simulink model "something_even_dumber"  (R2026b)
settings: Solver=ode23t  StopTime=simulation.timeSim  MaxStep=1/(5*solarPlant.converterSwitchingFrequency)  AbsTol=1e-3
PreLoadFcn:
  | run('something_dumb.mlx');
values from neighbouring files (symbols this model uses):
  Csc = Csc_cell/Ns_sc*Np_sc    (= 200)    [LunarDAB_Params.m]
  eta_sc = 0.95    [LunarDAB_Params.m]
  fsw = 100e3    (= 100000)    [LunarDAB_Params.m]
  k_restore = 1    [LunarDAB_Params.m]
  kiCurrent = 2    [LunarDAB_Params.m]
  kiVoltage = 8    [LunarDAB_Params.m]
  kpCurrent = 0.005    [LunarDAB_Params.m]
  kpVoltage = 0.4    [LunarDAB_Params.m]
  lTotal = lSeries + Llk    [LunarDAB_Params.m]
  P170_Imp = im(ix)    [P170_PV_Initialize.m]
  P170_Vmp = vm(ix)    [P170_PV_Initialize.m]
  Rd_bat = dV_droop/Ibat_max    (= 0.232258064516)    [LunarDAB_Params.m]
  SC_enable = 1    [LunarDAB_Params.m]
  thetaMaxDab = pi/4    (= 0.785398163397)    [LunarDAB_Params.m]
  Tsw = 1/fsw    (= 1e-05)    [LunarDAB_Params.m]
  Vsc0 = sqrt((Vsc_max^2 + Vsc_min^2)/2)    [LunarDAB_Params.m]
  Vsc_max = 119    [LunarDAB_Params.m]
  Vsc_min = 66    [LunarDAB_Params.m]
undefined symbols (not defined in the file or in its folder): a_lpf_sys, battery, bms, connectedLoad, dcVoltage, eta_dab, Ibat_sign, lunarCase, maxSoC, maxVdc, minIrrad, minSoC, minVdc, Ndab, olTime, P170_T, sc, sensor, solarPlant
libraries: nesl_utility x13, fl_lib x12, simulink x7, slpidlib x2, batteryecm_lib x1, simulink_extras x1, ee_lib x1
settings Model: Creator=The MathWorks, Inc.  LastModifiedBy=aj26g
settings SolverCC: AutoScaleAbsTol=off
settings DataIOCC: DSMLogging=off  ReturnWorkspaceOutputs=off  SaveOutput=off  SaveTime=off  SignalLoggingName=SolarPVDCWithBattery_logDB
settings OptimizationCC: ReuseModelBlockBuffer=off
settings DebuggingCC: SymbolicDimsDataTypeCodeGenerationDiagnostic=none  UnderSpecifiedDimensionMsg=warning
settings SFSimCC: CustomCodeUndefinedFunction=UseInterfaceOnly
settings RTWCC: DLArmComputeVersion=19.05
settings SimscapeCC: SimscapeLogName=simlog_SolarPVDCWithBattery  SimscapeLogSimulationStatistics=on  SimscapeLogType=all  SimscapeUseEnergyAccounting=off

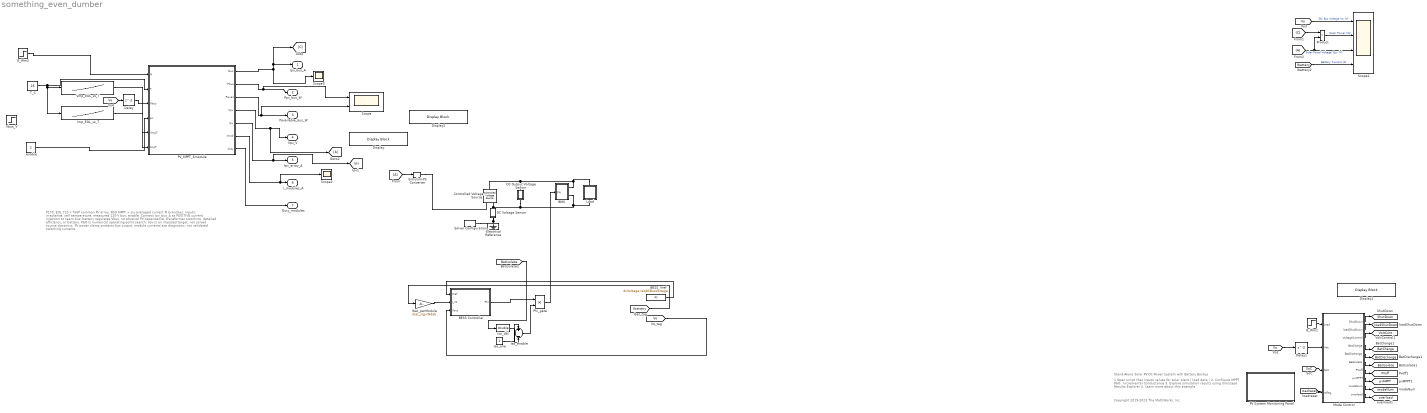
== system something_even_dumber ==
  note: 1 Open script that inputs values for solar plant ( load data )
      | 2. Configure MPPT P&O , Incremental Conductance
      | 3. Explore simulation results using Simscape Results Explorer
      | 4. Learn more about this example
  note: Stand-Alone Solar PV DC Power System with Battery Backup
  note: Copyright 2019-2023 The MathWorks, Inc.
  note: P170: EOL 72S x 756P common PV array. P&O MPPT + six averaged current PI branches.
      | Inputs: irradiance, cell temperature, measured 120-V bus, enable.
      | Connect Ipv_bus_A as POSITIVE current injection to team bus; battery regulates Vbus.
      |
      | no physical PV capacitance, transformer switching, detailed efficiency, or battery.
      | P&O is numerical operating-point search; Vpv is an imposed target, not solved source dynamics.
      | PV power clamp protects bus output; module currents are diagnostic, not validated switching currents.
  BESS Controller : Subsystem
  BESS_Vref : Constant  Value=dcVoltage.reqDCBusVoltage
  BMS : Subsystem
  Controlled Voltage Source : fl_lib/Electrical/Electrical Sources/Controlled Voltage Source
  DC Output Voltage Sensor : Subsystem
      mask Display: disp('v')
  DC Voltage Sensor : Subsystem
      mask Display: disp('v');
  Delay : Delay
  Delay1 : Delay
  Display : DisplayBlock  LabelPosition=Hide  Transparency=1  GridColor=[0.502, 0.502, 0.502]
  Display1 : DisplayBlock  LabelPosition=Hide  Transparency=1  GridColor=[0.502, 0.502, 0.502]
  Display2 : DisplayBlock  LabelPosition=Hide  Transparency=1  GridColor=[0.502, 0.502, 0.502]
  Electrical Reference : fl_lib/Electrical/Electrical Elements/Electrical Reference
  From : From
  From2 : From
  G_Wm1 : Step  Time=0.8  InitialValue=1367  FinalValue=700  SampleTime=0
  G_Wm2 : Step  Time=0.8  InitialValue=1367  FinalValue=700  SampleTime=0
  Goto2 : Goto
  Ibat_perModule : Gain  Gain=Ibat_sign/Ndab
  Imp_EOL_vs_T : Lookup_n-D  NumberOfTableDimensions=1  BreakpointsForDimension1=P170_T  Table=P170_Imp  InternalRulePriority=Speed  RndMeth=Simplest
  Iso_dbl : DataTypeConversion  OutDataTypeStr=double  SaturateOnIntegerOverflow=off  RndMeth=Floor
  Iso_enable : Sum  Inputs=+-
  Iso_one : Constant
  Load : Subsystem
  Mode Control : Stateflow chart  TreatAsAtomicUnit=on
  PV System Monitoring Panel : Subsystem
  PV_MPPT_6module : MATLAB Function  TreatAsAtomicUnit=on
  Phi_gate : Product
  Product : Product
  Scope : Scope  NumInputPorts=2
      settings: ActiveDisplayYMinimum=-1.4996053799360058  ActiveDisplayYMaximum=1.4239551585454688
  Scope1 : Scope  NumInputPorts=4
      settings: TimeSpan=simulation.timeSim  ActiveDisplayYMinimum=-72.27632  ActiveDisplayYMaximum=650.48692
  Scope2 : Scope
      settings: ActiveDisplayYMinimum=23.015586565193445  ActiveDisplayYMaximum=103.20798780153326  DataLoggingVariableName=ScopeData3
  Scope3 : Scope
      settings: ActiveDisplayYMinimum=-232.45862894967161  ActiveDisplayYMaximum=949.55274949917839  DataLoggingVariableName=ScopeData2
  Simulink-PS Converter : nesl_utility/Simulink-PS Converter  PhysicalDomain=network_engine_domain  SubClassName=ps_input  LeftPortType=input  RightPortType=output  PseudoPeriodic=off  Frequencies=[]  NoiseDistribution=none  NoiseParameters=[]  Unit=1  AffineConversion=off  FilteringAndDerivatives=provide  SimscapeFilterOrder=1  InputFilterTimeConstant=0.001  UdotUserProvided=0
  Solver Configuration : nesl_utility/Solver Configuration  PhysicalDomain=network_engine_domain  SubClassName=solver  LeftPortType=input  RightPortType=generic  Tones=[]  Harmonics=[]  SimulateNoise=off  Profile=off  UseLocalSampling=off  EnableSwitchedLinearOptims=on  FrequencyDomain=off  UseCCode=off  RelTol=0.001  AbsTol=1e-06  MinStep=1e-09  ToWorkspace=off  RevertToSquareIcSolve=off  NumHomotopyIterations=100  PhasorMode=off  PhasorModeNumHarmonics=1  ConsistencySolver=NEWTON_FTOL  CanonicalOrdering=UNORDERED  OptimizeIntermediates=UNOPTIMIZED  MulticoreSolverChoice=BACKWARD_EULER  IndexReductionMethod=DerivativeReplacement  DoDC=off  ResidualTolerance=1e-9  ConsistencyTolSource=GLOBAL  ConsistencyAbsTol=0.001  ConsistencyRelTol=0.001  ConsistencyTolFactor=0.001  UseLocalSolver=off  LocalSolverChoice=NE_TRAPEZOIDAL_ADVANCER  ResolveIndetEquations=on  FunctionEvalNumThread=1  LocalSolverSampleTime=2e-6  DoFixedCost=off  MaxNonlinIter=10  MaxModeIter=2  ComputeImpulses=off  ImpulseIterations=2  LinearAlgebra=auto  LinearAlgebraNumThread=0  EquationFormulation=NE_TIME_EF  DelaysMemoryBudget=1024  AutomaticFiltering=on  FilteringTimeConstant=0.001  PartitionStorageMethod=AS_NEEDED  PartitionMemoryBudget=1024  PartitionMethod=FAST  MultibodyUseLocalSolver=off  MultibodyLocalSolverChoice=ODE1  MultibodyLocalSolverSampleTime=0.001
  T_C : Constant  Value=25
  Vbus_V : Step  Time=1.2  InitialValue=120  FinalValue=115  SampleTime=0
  Vmp_EOL_vs_T : Lookup_n-D  NumberOfTableDimensions=1  BreakpointsForDimension1=P170_T  Table=P170_Vmp  InternalRulePriority=Speed  RndMeth=Simplest
  enable : Constant
  Ipv_bus_A : Outport
  Ppv_bus_W : Outport  Port=2
  Pavailable_bus_W : Outport  Port=3
  Vpv_V : Outport  Port=4
  Ipv_array_A : Outport  Port=5
  I_modules_A : Outport  Port=6
  Duty_modules : Outport  Port=7
  tag scope: BatCharge=global, BatDischarge=global, BatIsolate=global, Ipv=global, PVoff=global, ShutDown=global, VoltCont=global, loadShutDown=global, modeNum=global, overload=global, pvMPPT=global
  wires:
  Mode Control/5(BatDischarge) -> [BatDischarge]
  From2/1 -> Scope1/3, Product/2  "Solar Panel Voltage Vpv (V)"
  Product/1 -> Scope1/2  "Solar Power (W)"
  Mode Control/2(loadShutDown) -> [loadShutDown]
  Mode Control/9(modeNum) -> [modeNum]
  Mode Control/10(overload) -> [overload]
  [C] -> Product/1
  Mode Control/1(ShutDown) -> [ShutDown]
  Mode Control/3(VoltageControl) -> [VoltCont]
  Mode Control/8(pvMPPT) -> [pvMPPT]
  [loadreset] -> Mode Control/4(rsflag)
  [SoC] -> Mode Control/3(SoC)
  Mode Control/6(BatIsolate) -> [BatIsolate]
  G_Wm1/1 -> Mode Control/1(Irrad)
  Mode Control/7(PVoff) -> [PVoff]
  [Vo] -> Scope1/1  "DC Bus Voltage Vo (V)"
  Mode Control/4(BatCharge) -> [BatCharge]
  [Ibattery] -> Scope1/4  "Battery Current (A)"
  PV_MPPT_6module/6(Imod) -> Scope2/1, I_modules_A/1
  PV_MPPT_6module/1(Ibus) -> Scope3/1, [C], Ipv_bus_A/1
  G_Wm2/1 -> PV_MPPT_6module/1(G)
  PV_MPPT_6module/4(Vpv) -> Goto2/1, Vpv_V/1
  PV_MPPT_6module/5(Ipv) -> [Ipv], Ipv_array_A/1
  PV_MPPT_6module/7(duty) -> Duty_modules/1
  Imp_EOL_vs_T/1 -> PV_MPPT_6module/6(ImpT)
  PV_MPPT_6module/3(Pavail) -> Scope/2, Pavailable_bus_W/1
  enable/1 -> PV_MPPT_6module/4(en)
  PV_MPPT_6module/2(Pbus) -> Scope/1, Ppv_bus_W/1
  T_C/1 -> Vmp_EOL_vs_T/1, Imp_EOL_vs_T/1, PV_MPPT_6module/2(T)
  Vmp_EOL_vs_T/1 -> PV_MPPT_6module/5(VmpT)
  From/1 -> Simulink-PS Converter/1
  Ibat_perModule/1 -> BESS Controller/2(I_V1)
  [BatIsolate] -> Iso_dbl/1
  Iso_enable/1 -> Phi_gate/2
  BESS_Vref/1 -> BESS Controller/1(Vref)
  [Vo] -> BESS Controller/3(Vout)
  [Ibattery] -> Ibat_perModule/1
  Phi_gate/1 -> BMS/1(Phi)
  Iso_one/1 -> Iso_enable/1
  Iso_dbl/1 -> Iso_enable/2
  BESS Controller/1(Phi) -> Phi_gate/1
  [Vo] -> Delay/1
  Delay/1 -> PV_MPPT_6module/3(Vbus)
  [Vo] -> Delay1/1
  Delay1/1 -> Mode Control/2(Vdc)
  connections:
  BMS/RConn1 -- Load/LConn1 -- DC Output Voltage Sensor/RConn1 -- Controlled Voltage Source/LConn1
  Solver Configuration/RConn1 -- Electrical Reference/LConn1 -- DC Voltage Sensor/LConn1
  Simulink-PS Converter/RConn1 -- Controlled Voltage Source/RConn1
  Load/RConn1 -- DC Output Voltage Sensor/LConn1 -- Controlled Voltage Source/RConn2 -- DC Voltage Sensor/RConn1 -- BMS/RConn2

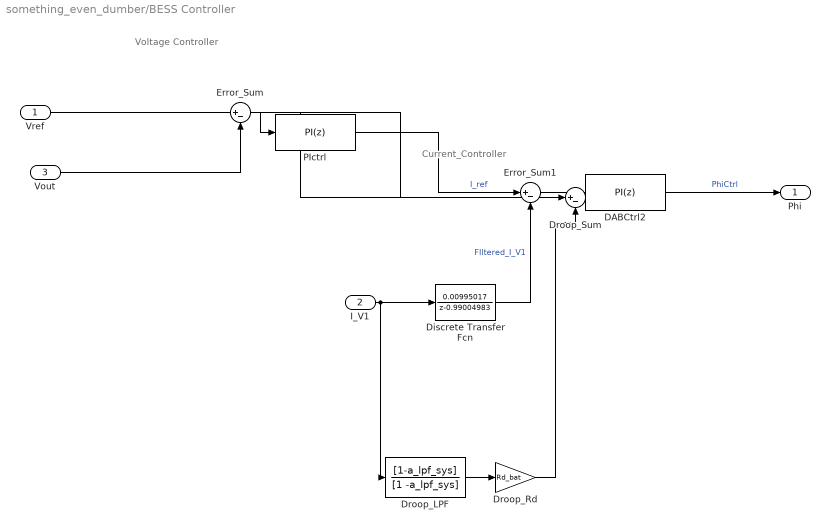
== system something_even_dumber/BESS Controller ==
  note: Current_Controller
  note: Voltage Controller
  Vref : Inport
  I_V1 : Inport  Port=2
  Vout : Inport  Port=3
  DABCtrl2 : slpidlib/PID Controller  Controller=PI  Form=Parallel  TimeDomain=Discrete-time  UseExternalTs=off  SampleTime=Tsw  IntegratorMethod=Forward Euler  FilterMethod=Forward Euler  ControllerParametersSource=internal  P=kpCurrent  I=kiCurrent  UseKiTs=off  D=0  UseExternalDerivativeSource=off  N=100  UseFilter=on  TunerSelectOption=Transfer Function Based (PID Tuner App)  InitialConditionSource=internal  InitialConditionForIntegrator=thetaIC  InitialConditionForFilter=0  DifferentiatorICPrevScaledInput=0  ExternalReset=none  TrackingMode=off  Kt=1  LimitOutput=on  SatLimitsSource=internal  UpperSaturationLimit=thetaMaxDab  LowerSaturationLimit=-thetaMaxDab  LinearizeAsGain=off  AntiWindupMode=none  Kb=1  LimitIntegrator=off  UpperIntegratorSaturationLimit=inf  LowerIntegratorSaturationLimit=-inf  RndMeth=Simplest  POutMin=[]  POutMax=[]  IOutMin=[]  IOutMax=[]  DOutMin=[]  DOutMax=[]  NOutMin=[]  NOutMax=[]  SumOutMin=[]  SumOutMax=[]  SaturationOutDataTypeStr=Inherit: Inherit via back propagation  SaturationOutMin=[]  SaturationOutMax=[]  PParamMin=[]  PParamMax=[]  IParamMin=[]  IParamMax=[]  DParamMin=[]  DParamMax=[]  NParamMin=[]  NParamMax=[]  KbParamMin=[]  KbParamMax=[]  KtParamMin=[]  KtParamMax=[]  KbOutMin=[]  KbOutMax=[]  KtOutMin=[]  KtOutMax=[]  IntegratorOutMin=[]  IntegratorOutMax=[]  FilterOutMin=[]  FilterOutMax=[]  SumI1OutMin=[]  SumI1OutMax=[]  SumI2OutMin=[]  SumI2OutMax=[]  SumI3OutMin=[]  SumI3OutMax=[]  SumI4OutMin=[]  SumI4OutMax=[]  SumDOutMin=[]  SumDOutMax=[]  DifferentiatorOutMin=[]  DifferentiatorOutMax=[]  FilterDiffOutCoefMin=[]  FilterDiffOutCoefMax=[]  ReciprocalOutMin=[]  ReciprocalOutMax=[]  SumDenOutMin=[]  SumDenOutMax=[]  SumNumOutMin=[]  SumNumOutMax=[]  DivideOutMin=[]  DivideOutMax=[]  UdiffTsProdOutMin=[]  UdiffTsProdOutMax=[]  NTsProdOutMin=[]  NTsProdOutMax=[]  UintegralTsProdOutMin=[]  UintegralTsProdOutMax=[]  UngainTsProdOutMin=[]  UngainTsProdOutMax=[]  ClampingZeroOutDataTypeStr=Inherit: Inherit via back propagation  ClampingZeroOutMin=[]  ClampingZeroOutMax=[]  FilterDenConstantOutDataTypeStr=Inherit: Inherit via back propagation  FilterDenConstantOutMin=[]  FilterDenConstantOutMax=[]  PCopyOutDataTypeStr=Inherit: Inherit via back propagation  PCopyOutMin=[]  PCopyOutMax=[]  NCopyOutDataTypeStr=Inherit: Inherit via back propagation  NCopyOutMin=[]  NCopyOutMax=[]  IntegratorContinuousStateAttributes=''  IntegratorStateMustResolveToSignalObject=off  IntegratorRTWStateStorageClass=Auto  FilterContinuousStateAttributes=''  FilterStateMustResolveToSignalObject=off  FilterRTWStateStorageClass=Auto  ParallelPVariant=InternalParameters  IdealPVariant=Disabled  IVariant=InternalParameters  DVariant=Disabled  IntegratorVariant=Discrete  SatVariant=Enabled  AWVariant=Passthrough  PCopyVariant=Disabled  TRVariant=Disabled  FdbkBlocksVariant=Forward  IdealPFdbkVariant=Disabled  SatFdbkVariant=Disabled  DerivativeFilterVariant=Disabled  NVariant=Disabled  NCopyVariant=Disabled_SignalSpec  FilterICVariant=Disabled  IntegratorICVariant=InternalICs  ExternalResetVariant=Disabled  TRSumVariant=Passthrough  SumFdbkVariant=Disabled  SumVariant=Sum_PI  TsampFilterVariant=InternalTs  TsampNgainVariant=Passthrough  TsampIntegralVariant=Disabled_SignalSpec  ExternalSaturationOutDataTypeStr=Inherit: Same as second input  DerivativeSourceVariant=Disabled  PreIntVariant=InternalPreInt
      settings: LibrarySourceBlock=mcblib/Control/Synchronous Machine/Controllers/PI Controller
  Discrete Transfer Fcn : DiscreteTransferFcn  Numerator=[0.00995017]  Denominator=[1 -0.99004983]
  Droop_LPF : DiscreteTransferFcn  Numerator=[1-a_lpf_sys]  Denominator=[1 -a_lpf_sys]  SampleTime=Tsw
  Droop_Rd : Gain  Gain=Rd_bat
  Droop_Sum : Sum  Inputs=|+-
  Error_Sum : Sum  Inputs=|+-
  Error_Sum1 : Sum  Inputs=|+-
  PIctrl : slpidlib/PID Controller  Controller=PI  Form=Parallel  TimeDomain=Discrete-time  UseExternalTs=off  SampleTime=Tsw  IntegratorMethod=Forward Euler  FilterMethod=Forward Euler  ControllerParametersSource=internal  P=kpVoltage  I=kiVoltage  UseKiTs=off  D=0  UseExternalDerivativeSource=off  N=100  UseFilter=on  TunerSelectOption=Transfer Function Based (PID Tuner App)  InitialConditionSource=internal  InitialConditionForIntegrator=thetaIC  InitialConditionForFilter=0  DifferentiatorICPrevScaledInput=0  ExternalReset=none  TrackingMode=off  Kt=1  LimitOutput=on  SatLimitsSource=internal  UpperSaturationLimit=45  LowerSaturationLimit=-45  LinearizeAsGain=off  AntiWindupMode=none  Kb=1  LimitIntegrator=off  UpperIntegratorSaturationLimit=inf  LowerIntegratorSaturationLimit=-inf  RndMeth=Simplest  POutMin=[]  POutMax=[]  IOutMin=[]  IOutMax=[]  DOutMin=[]  DOutMax=[]  NOutMin=[]  NOutMax=[]  SumOutMin=[]  SumOutMax=[]  SaturationOutDataTypeStr=Inherit: Inherit via back propagation  SaturationOutMin=[]  SaturationOutMax=[]  PParamMin=[]  PParamMax=[]  IParamMin=[]  IParamMax=[]  DParamMin=[]  DParamMax=[]  NParamMin=[]  NParamMax=[]  KbParamMin=[]  KbParamMax=[]  KtParamMin=[]  KtParamMax=[]  KbOutMin=[]  KbOutMax=[]  KtOutMin=[]  KtOutMax=[]  IntegratorOutMin=[]  IntegratorOutMax=[]  FilterOutMin=[]  FilterOutMax=[]  SumI1OutMin=[]  SumI1OutMax=[]  SumI2OutMin=[]  SumI2OutMax=[]  SumI3OutMin=[]  SumI3OutMax=[]  SumI4OutMin=[]  SumI4OutMax=[]  SumDOutMin=[]  SumDOutMax=[]  DifferentiatorOutMin=[]  DifferentiatorOutMax=[]  FilterDiffOutCoefMin=[]  FilterDiffOutCoefMax=[]  ReciprocalOutMin=[]  ReciprocalOutMax=[]  SumDenOutMin=[]  SumDenOutMax=[]  SumNumOutMin=[]  SumNumOutMax=[]  DivideOutMin=[]  DivideOutMax=[]  UdiffTsProdOutMin=[]  UdiffTsProdOutMax=[]  NTsProdOutMin=[]  NTsProdOutMax=[]  UintegralTsProdOutMin=[]  UintegralTsProdOutMax=[]  UngainTsProdOutMin=[]  UngainTsProdOutMax=[]  ClampingZeroOutDataTypeStr=Inherit: Inherit via back propagation  ClampingZeroOutMin=[]  ClampingZeroOutMax=[]  FilterDenConstantOutDataTypeStr=Inherit: Inherit via back propagation  FilterDenConstantOutMin=[]  FilterDenConstantOutMax=[]  PCopyOutDataTypeStr=Inherit: Inherit via back propagation  PCopyOutMin=[]  PCopyOutMax=[]  NCopyOutDataTypeStr=Inherit: Inherit via back propagation  NCopyOutMin=[]  NCopyOutMax=[]  IntegratorContinuousStateAttributes=''  IntegratorStateMustResolveToSignalObject=off  IntegratorRTWStateStorageClass=Auto  FilterContinuousStateAttributes=''  FilterStateMustResolveToSignalObject=off  FilterRTWStateStorageClass=Auto  ParallelPVariant=InternalParameters  IdealPVariant=Disabled  IVariant=InternalParameters  DVariant=Disabled  IntegratorVariant=Discrete  SatVariant=Enabled  AWVariant=Passthrough  PCopyVariant=Disabled  TRVariant=Disabled  FdbkBlocksVariant=Forward  IdealPFdbkVariant=Disabled  SatFdbkVariant=Disabled  DerivativeFilterVariant=Disabled  NVariant=Disabled  NCopyVariant=Disabled_SignalSpec  FilterICVariant=Disabled  IntegratorICVariant=InternalICs  ExternalResetVariant=Disabled  TRSumVariant=Passthrough  SumFdbkVariant=Disabled  SumVariant=Sum_PI  TsampFilterVariant=InternalTs  TsampNgainVariant=Passthrough  TsampIntegralVariant=Disabled_SignalSpec  ExternalSaturationOutDataTypeStr=Inherit: Same as second input  DerivativeSourceVariant=Disabled  PreIntVariant=InternalPreInt
      settings: LibrarySourceBlock=mcblib/Control/Synchronous Machine/Controllers/PI Controller
  Phi : Outport
  wires:
  Error_Sum/1 -> PIctrl/1
  PIctrl/1 -> Error_Sum1/1  "I_ref"
  Vout/1 -> Error_Sum/2
  Error_Sum1/1 -> DABCtrl2/1
  DABCtrl2/1 -> Phi/1  "PhiCtrl"
  I_V1/1 -> Discrete Transfer Fcn/1, Droop_LPF/1
  Discrete Transfer Fcn/1 -> Error_Sum1/2  "FIltered_I_V1"
  Vref/1 -> Droop_Sum/1
  Droop_LPF/1 -> Droop_Rd/1
  Droop_Rd/1 -> Droop_Sum/2
  Droop_Sum/1 -> Error_Sum/1

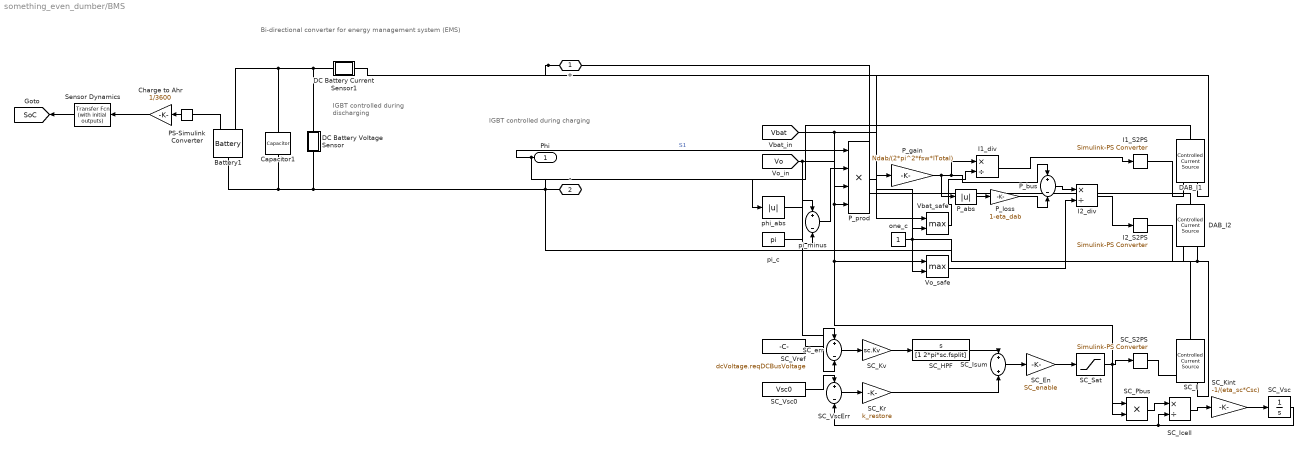
== system something_even_dumber/BMS ==
  note: IGBT controlled during charging
  note: Bi-directional converter for energy management system (EMS)
  note: IGBT controlled during discharging
  Phi : Inport
  Battery1 : batteryecm_lib/Battery  Vnom=battery.nominalBatteryVoltage V  prm_dir=1  R1_dis=2 Ohm  R1_ch=2 Ohm  R1=0.01 Ohm  prm_AH=2  AH=connectedLoad.batteryAmpHr hr*A  V1=battery.minBatteryNominalVoltage V  AH1=connectedLoad.batteryAmpHr*0.2 hr*A  prm_R2=2  R2=2000 Ohm  Tmeas=298.15 K  charge_measurement_port=simscape.enum.battery.enable.yes  prm_dyn=1  Rp1=0.005 Ohm  tau1=30 s  Rp2=0.005 Ohm  tau2=30 s  Rp3=0.005 Ohm  tau3=30 s  Rp4=0.005 Ohm  tau4=30 s  Rp5=0.005 Ohm  tau5=30 s  prm_fade=1  N_fade=100  AH_fade=45 hr*A  R1_fade=2.02 Ohm  R1_ch_fade=2.02 Ohm  V1_fade=10.35 V  prm_age=1  prm_age_OCV=1  OCV_age=0.9  SOC_age=60  Tmeas_age=298.15 K  delta_time_age_vec=[0] d  temperature_age_vec=[273] K  OCV_scaling_age=2.2134e6  OCV_offset_age=1.632e6  temp_exp_age=0.515833569 V  t_exp_age=0.75  Vnom_T2=12 V  R1_T2=2.2 Ohm  R1_T2_dis=2.2 Ohm  R1_T2_ch=2.2 Ohm  V1_T2=11.4 V  R2_T2=2200 Ohm  Rp1_T2=0.005 Ohm  tau1_T2=30 s  Rp2_T2=0.005 Ohm  tau2_T2=30 s  Rp3_T2=0.005 Ohm  tau3_T2=30 s  Rp4_T2=0.005 Ohm  tau4_T2=30 s  Rp5_T2=0.005 Ohm  tau5_T2=30 s  Tmeas2=273.15 K  thermal_port=simscape.enum.thermaleffects.omit  thermal_mass=30000 J/K  i_specify=off  i_priority=None  i=0 A  i_nominal_specify=off  i_nominal_value=1  i_nominal_unit=A  v_specify=off  v_priority=None  v=0 V  v_nominal_specify=off  v_nominal_value=1  v_nominal_unit=V  charge_specify=on  charge_priority=High  charge=batteryInitialStateOfCharge hr*A  charge_nominal_specify=off  charge_nominal_value=1  charge_nominal_unit=A*hr  num_cycles_specify=off  num_cycles_priority=High  num_cycles=0  num_cycles_nominal_specify=off  num_cycles_nominal_value=1  num_cycles_nominal_unit=1  temperature_specify=off  temperature_priority=High  temperature=298.15 K  temperature_nominal_specify=off  temperature_nominal_value=1  temperature_nominal_unit=K
  Capacitor1 : fl_lib/Electrical/Electrical Elements/Capacitor  c=boost.outputCapacitor F  r=1e-6 Ohm  g=0 1/Ohm  i_specify=off  i_priority=None  i=0 A  i_nominal_specify=off  i_nominal_value=1  i_nominal_unit=A  v_specify=off  v_priority=None  v=0 V  v_nominal_specify=off  v_nominal_value=1  v_nominal_unit=V  vc_specify=on  vc_priority=High  vc=batteryInputCapacitorInitialVoltage V  vc_nominal_specify=off  vc_nominal_value=1  vc_nominal_unit=V
  Charge to Ahr : Gain  Gain=1/3600
  DAB_I1 : fl_lib/Electrical/Electrical Sources/Controlled Current Source
  DAB_I2 : fl_lib/Electrical/Electrical Sources/Controlled Current Source
  DC Battery Current Sensor1 : Subsystem
      mask Display: disp('i');
  DC Battery Voltage Sensor : Subsystem
      mask Display: disp('v');
  I1_S2PS : nesl_utility/Simulink-PS Converter  PhysicalDomain=network_engine_domain  SubClassName=ps_input  LeftPortType=input  RightPortType=output  PseudoPeriodic=off  Frequencies=[]  NoiseDistribution=none  NoiseParameters=[]  Unit=1  AffineConversion=off  FilteringAndDerivatives=provide  SimscapeFilterOrder=1  InputFilterTimeConstant=0.001  UdotUserProvided=0
  I1_div : Product  Inputs=*/
  I2_S2PS : nesl_utility/Simulink-PS Converter  PhysicalDomain=network_engine_domain  SubClassName=ps_input  LeftPortType=input  RightPortType=output  PseudoPeriodic=off  Frequencies=[]  NoiseDistribution=none  NoiseParameters=[]  Unit=1  AffineConversion=off  FilteringAndDerivatives=provide  SimscapeFilterOrder=1  InputFilterTimeConstant=0.001  UdotUserProvided=0
  I2_div : Product  Inputs=*/
  PS-Simulink Converter : nesl_utility/PS-Simulink Converter  PhysicalDomain=network_engine_domain  SubClassName=ps_output  LeftPortType=input  RightPortType=output  PseudoPeriodic=off  Frequencies=[]  VectorFormat=1-D array  Unit=inherit  AffineConversion=off
  P_abs : Abs  SaturateOnIntegerOverflow=off
  P_bus : Sum  Inputs=+-
  P_gain : Gain  Gain=Ndab/(2*pi^2*fsw*lTotal)
  P_loss : Gain  Gain=1-eta_dab
  P_prod : Product  Inputs=4
  SC_En : Gain  Gain=SC_enable
  SC_HPF : TransferFcn  Numerator=[1 0]  Denominator=[1 2*pi*sc.fsplit]
  SC_I : fl_lib/Electrical/Electrical Sources/Controlled Current Source
  SC_Icell : Product  Inputs=*/
  SC_Isum : Sum
  SC_Kint : Gain  Gain=-1/(eta_sc*Csc)
  SC_Kr : Gain  Gain=k_restore
  SC_Kv : Gain  Gain=sc.Kv
  SC_Pbus : Product
  SC_S2PS : nesl_utility/Simulink-PS Converter  PhysicalDomain=network_engine_domain  SubClassName=ps_input  LeftPortType=input  RightPortType=output  PseudoPeriodic=off  Frequencies=[]  NoiseDistribution=none  NoiseParameters=[]  Unit=1  AffineConversion=off  FilteringAndDerivatives=provide  SimscapeFilterOrder=1  InputFilterTimeConstant=0.001  UdotUserProvided=0
  SC_Sat : Saturate  UpperLimit=sc.Imax  LowerLimit=-sc.Imax
  SC_Vref : Constant  Value=dcVoltage.reqDCBusVoltage
  SC_Vsc : Integrator  InitialCondition=Vsc0  LimitOutput=on  UpperSaturationLimit=Vsc_max  LowerSaturationLimit=Vsc_min
  SC_Vsc0 : Constant  Value=Vsc0
  SC_VscErr : Sum  Inputs=+-
  SC_err : Sum  Inputs=+-
  Sensor Dynamics : simulink_extras/Additional Linear/Transfer Fcn (with initial outputs)  N=[1]  D=[1/sensor.samplingFreq 1]  Y0=minSoC  U0=0
  Vbat_safe : MinMax  Function=max  Inputs=2
  Vo_safe : MinMax  Function=max  Inputs=2
  one_c : Constant
  phi_abs : Abs  SaturateOnIntegerOverflow=off
  pi_c : Constant  Value=pi
  pi_minus : Sum  Inputs=+-
  + : PMIOPort  Side=Right
  - : PMIOPort  Port=2  Side=Right
  tag scope: SoC=global
  wires:
  PS-Simulink Converter/1 -> Charge to Ahr/1
  Sensor Dynamics/1 -> [SoC]
  Charge to Ahr/1 -> Sensor Dynamics/1
  Phi/1 -> phi_abs/1, P_prod/1  "S1"
  pi_c/1 -> pi_minus/1
  phi_abs/1 -> pi_minus/2
  pi_minus/1 -> P_prod/2
  [Vbat] -> P_prod/3, Vbat_safe/1
  [Vo] -> Vo_safe/1, SC_Pbus/2, P_prod/4, SC_err/2
  P_prod/1 -> P_gain/1
  one_c/1 -> Vbat_safe/2, Vo_safe/2
  P_gain/1 -> I1_div/1, P_bus/1, P_abs/1
  Vbat_safe/1 -> I1_div/2
  P_abs/1 -> P_loss/1
  P_loss/1 -> P_bus/2
  P_bus/1 -> I2_div/1
  Vo_safe/1 -> I2_div/2
  SC_Vref/1 -> SC_err/1
  SC_err/1 -> SC_Kv/1
  SC_Kv/1 -> SC_HPF/1
  SC_Vsc0/1 -> SC_VscErr/1
  SC_Vsc/1 -> SC_VscErr/2, SC_Icell/2
  SC_VscErr/1 -> SC_Kr/1
  SC_HPF/1 -> SC_Isum/1
  SC_Kr/1 -> SC_Isum/2
  SC_Isum/1 -> SC_En/1
  SC_En/1 -> SC_Sat/1
  SC_Sat/1 -> SC_Pbus/1, SC_S2PS/1
  SC_Pbus/1 -> SC_Icell/1
  SC_Icell/1 -> SC_Kint/1
  SC_Kint/1 -> SC_Vsc/1
  I1_div/1 -> I1_S2PS/1
  I2_div/1 -> I2_S2PS/1
  connections:
  Battery1/RConn1 -- Capacitor1/RConn1 -- DC Battery Voltage Sensor/LConn1 -- SC_I/RConn2 -- DAB_I2/RConn2 -- -/RConn1 -- DAB_I1/LConn1
  Battery1/LConn2 -- PS-Simulink Converter/LConn1
  DC Battery Current Sensor1/LConn1 -- DC Battery Voltage Sensor/RConn1 -- Battery1/LConn1 -- Capacitor1/LConn1
  I1_S2PS/RConn1 -- DAB_I1/RConn1
  I2_S2PS/RConn1 -- DAB_I2/RConn1
  SC_S2PS/RConn1 -- SC_I/RConn1
  DAB_I1/RConn2 -- DC Battery Current Sensor1/RConn1
  +/RConn1 -- DAB_I2/LConn1 -- SC_I/LConn1

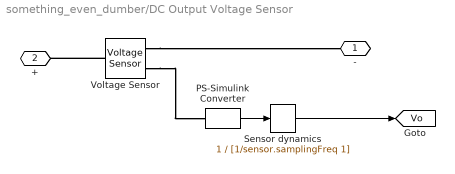
== system something_even_dumber/DC Output Voltage Sensor ==
  PS-Simulink Converter : nesl_utility/PS-Simulink Converter  PhysicalDomain=network_engine_domain  SubClassName=ps_output  LeftPortType=input  RightPortType=output  PseudoPeriodic=off  Frequencies=[]  VectorFormat=1-D array  Unit=1  AffineConversion=off
  Sensor dynamics : TransferFcn  Numerator=1  Denominator=[1/sensor.samplingFreq 1]
  Voltage Sensor : fl_lib/Electrical/Electrical Sensors/Voltage Sensor
  - : PMIOPort  Side=Left
  + : PMIOPort  Port=2  Side=Right
  tag scope: Vo=global
  wires:
  PS-Simulink Converter/1 -> Sensor dynamics/1
  Sensor dynamics/1 -> [Vo]
  connections:
  Voltage Sensor/RConn2 -- -/RConn1
  Voltage Sensor/RConn1 -- PS-Simulink Converter/LConn1
  Voltage Sensor/LConn1 -- +/RConn1

== system something_even_dumber/DC Voltage Sensor ==
  PS-Simulink Converter : nesl_utility/PS-Simulink Converter  PhysicalDomain=network_engine_domain  SubClassName=ps_output  LeftPortType=input  RightPortType=output  PseudoPeriodic=off  Frequencies=[]  VectorFormat=1-D array  Unit=1  AffineConversion=off
  Sensor dynamics : TransferFcn  Numerator=1  Denominator=[1/sensor.samplingFreq 1]
  Voltage Sensor : fl_lib/Electrical/Electrical Sensors/Voltage Sensor
      settings: LogSimulationData=on
  - : PMIOPort  Side=Left
  + : PMIOPort  Port=2  Side=Right
  tag scope: Vpv=global
  wires:
  PS-Simulink Converter/1 -> Sensor dynamics/1
  Sensor dynamics/1 -> [Vpv]
  connections:
  Voltage Sensor/LConn1 -- +/RConn1
  Voltage Sensor/RConn1 -- PS-Simulink Converter/LConn1
  Voltage Sensor/RConn2 -- -/RConn1

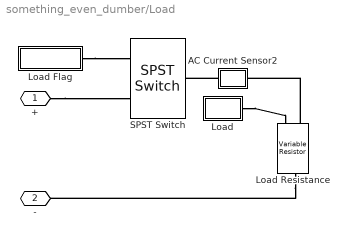
== system something_even_dumber/Load ==
  AC Current Sensor2 : Subsystem
      mask Display: disp('i');
  Load : Subsystem
  Load Flag : Subsystem
  Load Resistance : fl_lib/Electrical/Electrical Elements/Variable Resistor  Rmin=0 Ohm  thermalEnable=false  thermal_mass=1 J/K  i_specify=off  i_priority=None  i=5 A  i_nominal_specify=off  i_nominal_value=1  i_nominal_unit=A  v_specify=off  v_priority=None  v=0 V  v_nominal_specify=off  v_nominal_value=1  v_nominal_unit=V  T_specify=off  T_priority=None  T=300 K  T_nominal_specify=off  T_nominal_value=1  T_nominal_unit=K
  SPST Switch : ee_lib/Switches & Breakers/SPST Switch  R_closed=0.01 Ohm  G_open=1e-6 S  Threshold=0.5 V  Width=0 V  model_dynamics=0  t_on=1e-3 s  t_off=1e-3 s  initial_vT=0 V
  + : PMIOPort  Side=Left
  - : PMIOPort  Port=2  Side=Right
  connections:
  +/RConn1 -- SPST Switch/LConn2
  Load Resistance/LConn2 -- AC Current Sensor2/LConn1
  Load Resistance/RConn1 -- -/RConn1
  Load/RConn1 -- Load Resistance/LConn1
  Load Flag/RConn1 -- SPST Switch/LConn1
  AC Current Sensor2/RConn1 -- SPST Switch/RConn1

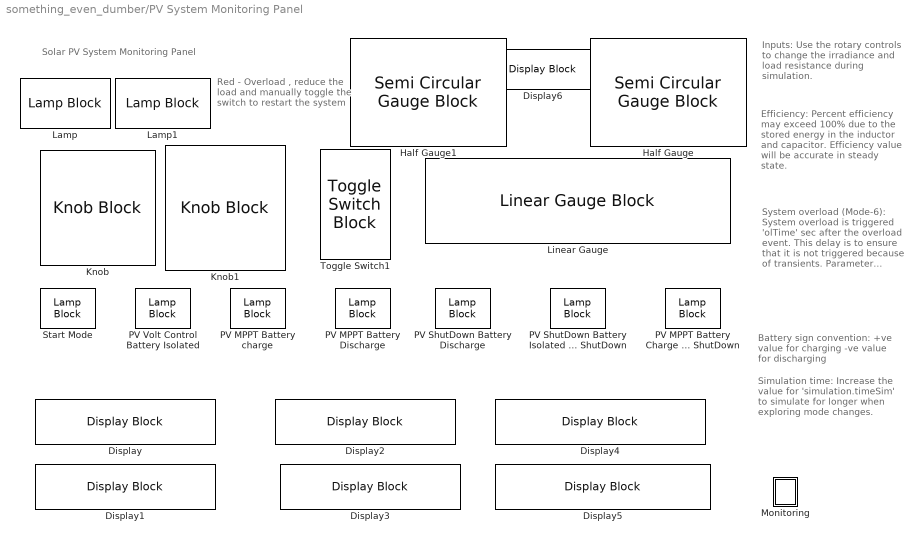
== system something_even_dumber/PV System Monitoring Panel ==
  note: Red - Overload , reduce the load and manually toggle the switch to restart the system
  note: Solar PV System Monitoring Panel
  note: Simulation time:
      | Increase the value for 'simulation.timeSim' to simulate for longer when exploring mode changes.
  note: Inputs:
      | Use the rotary controls to change the irradiance and load resistance during simulation.
  note: System overload (Mode-6):
      | System overload is triggered 'olTime' sec after the overload event. This delay is to ensure that it is not triggered because of transients. Parameter 'olTime' can be modified in the supporting livescript.
  note: Efficiency:
      | Percent efficiency may exceed 100% due to the stored energy in the inductor and capacitor. Efficiency value will be accurate in steady state.
  note: Battery sign convention:
      | +ve value for charging
      | -ve value for discharging
  Display{,1..6} (7 alike) : DisplayBlock  Transparency=1  GridColor=[0.502, 0.502, 0.502]
  Half Gauge : SemiCircularGaugeBlock  ScaleMin=20  FontColor=[0.0, 0.0, 0.0]
  Half Gauge1 : SemiCircularGaugeBlock  FontColor=[0.0, 0.0, 0.0]
  Knob : KnobBlock  ScaleMin=150  ScaleMax=1000
  Knob1 : KnobBlock  ScaleMin=0.15  ScaleMax=20
  Lamp : LampBlock  DefaultColor=[192.0, 192.0, 192.0]
  Lamp1 : LampBlock  DefaultColor=[192.0, 192.0, 192.0]
  Linear Gauge : LinearGaugeBlock  ScaleMin=-100  FontColor=[0.0, 0.0, 0.0]
  Monitoring : Subsystem
  PV MPPT Battery Charge Load ShutDown : LampBlock  DefaultColor=[192.0, 192.0, 192.0]
  PV MPPT Battery Discharge : LampBlock  DefaultColor=[192.0, 192.0, 192.0]
  PV MPPT Battery charge : LampBlock  DefaultColor=[192.0, 192.0, 192.0]
  PV ShutDown Battery Discharge : LampBlock  DefaultColor=[192.0, 192.0, 192.0]
  PV ShutDown Battery Isolated System ShutDown : LampBlock  DefaultColor=[192.0, 192.0, 192.0]
  PV Volt Control Battery Isolated : LampBlock  DefaultColor=[192.0, 192.0, 192.0]
  Start Mode : LampBlock  DefaultColor=[192.0, 192.0, 192.0]
  Toggle Switch1 : ToggleSwitchBlock

== system something_even_dumber/BMS/DC Battery Current Sensor1 ==
  Current Sensor : fl_lib/Electrical/Electrical Sensors/Current Sensor
  PS-Simulink Converter : nesl_utility/PS-Simulink Converter  PhysicalDomain=network_engine_domain  SubClassName=ps_output  LeftPortType=input  RightPortType=output  PseudoPeriodic=off  Frequencies=[]  VectorFormat=1-D array  Unit=1  AffineConversion=off
  Sensor dynamics : TransferFcn  Numerator=1  Denominator=[1/sensor.samplingFreq 1]
  - : PMIOPort  Side=Left
  + : PMIOPort  Port=2  Side=Right
  tag scope: Ibattery=global
  wires:
  PS-Simulink Converter/1 -> Sensor dynamics/1
  Sensor dynamics/1 -> [Ibattery]
  connections:
  Current Sensor/RConn1 -- PS-Simulink Converter/LConn1
  +/RConn1 -- Current Sensor/LConn1
  Current Sensor/RConn2 -- -/RConn1

== system something_even_dumber/BMS/DC Battery Voltage Sensor ==
  PS-Simulink Converter : nesl_utility/PS-Simulink Converter  PhysicalDomain=network_engine_domain  SubClassName=ps_output  LeftPortType=input  RightPortType=output  PseudoPeriodic=off  Frequencies=[]  VectorFormat=1-D array  Unit=1  AffineConversion=off
  Sensor dynamics : TransferFcn  Numerator=1  Denominator=[1/sensor.samplingFreq 1]
  Voltage Sensor : fl_lib/Electrical/Electrical Sensors/Voltage Sensor
      settings: LogSimulationData=on
  - : PMIOPort  Side=Left
  + : PMIOPort  Port=2  Side=Right
  tag scope: Vbat=global
  wires:
  PS-Simulink Converter/1 -> Sensor dynamics/1
  Sensor dynamics/1 -> [Vbat]
  connections:
  Voltage Sensor/LConn1 -- +/RConn1
  Voltage Sensor/RConn1 -- PS-Simulink Converter/LConn1
  Voltage Sensor/RConn2 -- -/RConn1

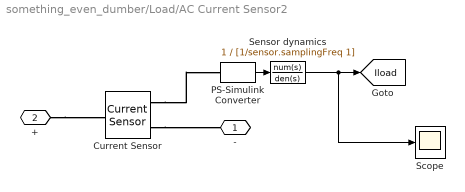
== system something_even_dumber/Load/AC Current Sensor2 ==
  Current Sensor : fl_lib/Electrical/Electrical Sensors/Current Sensor
  PS-Simulink Converter : nesl_utility/PS-Simulink Converter  PhysicalDomain=network_engine_domain  SubClassName=ps_output  LeftPortType=input  RightPortType=output  PseudoPeriodic=off  Frequencies=[]  VectorFormat=1-D array  Unit=1  AffineConversion=off
  Scope : Scope
      settings: ActiveDisplayYMinimum=-2.69141  ActiveDisplayYMaximum=24.19807  DataLoggingVariableName=ScopeData4
  Sensor dynamics : TransferFcn  Numerator=1  Denominator=[1/sensor.samplingFreq 1]
  - : PMIOPort  Side=Left
  + : PMIOPort  Port=2  Side=Right
  tag scope: Iload=global
  wires:
  PS-Simulink Converter/1 -> Sensor dynamics/1
  Sensor dynamics/1 -> Scope/1, [Iload]
  connections:
  Current Sensor/RConn1 -- PS-Simulink Converter/LConn1
  +/RConn1 -- Current Sensor/LConn1
  Current Sensor/RConn2 -- -/RConn1

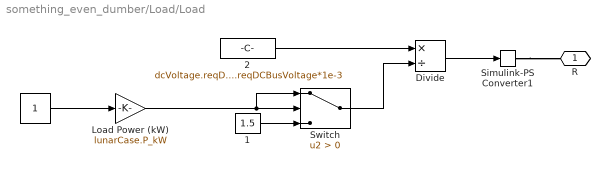
== system something_even_dumber/Load/Load ==
  " " : Constant
  " 1" : Constant  Value=1.5
  " 2" : Constant  Value=dcVoltage.reqDCBusVoltage*dcVoltage.reqDCBusVoltage*1e-3
  Divide : Product  Inputs=*/
  Load Power (kW) : Gain  Gain=lunarCase.P_kW
  Simulink-PS Converter1 : nesl_utility/Simulink-PS Converter  PhysicalDomain=network_engine_domain  SubClassName=ps_input  LeftPortType=input  RightPortType=output  PseudoPeriodic=off  Frequencies=[]  NoiseDistribution=none  NoiseParameters=[]  Unit=1  AffineConversion=off  FilteringAndDerivatives=provide  SimscapeFilterOrder=1  InputFilterTimeConstant=0.001  UdotUserProvided=0
  Switch : Switch  Criteria=u2 > Threshold  SaturateOnIntegerOverflow=off  InputSameDT=off
  R : PMIOPort  Side=Right
  wires:
  " "/1 -> Load Power (kW)/1
  Load Power (kW)/1 -> Switch/1, Switch/2
  " 1"/1 -> Switch/3
  " 2"/1 -> Divide/1
  Switch/1 -> Divide/2
  Divide/1 -> Simulink-PS Converter1/1
  connections:
  Simulink-PS Converter1/RConn1 -- R/RConn1

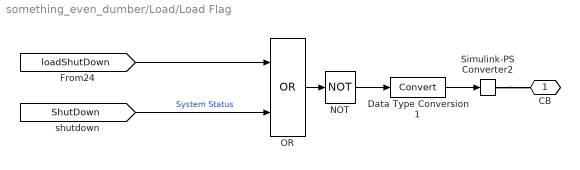
== system something_even_dumber/Load/Load Flag ==
  Data Type Conversion1 : DataTypeConversion  SaturateOnIntegerOverflow=off  RndMeth=Floor
  NOT : Logic  Operator=NOT  IconShape=distinctive  AllPortsSameDT=off  OutDataTypeStr=boolean
  OR : Logic  Operator=OR  IconShape=distinctive  AllPortsSameDT=off  OutDataTypeStr=boolean
  Simulink-PS Converter2 : nesl_utility/Simulink-PS Converter  PhysicalDomain=network_engine_domain  SubClassName=ps_input  LeftPortType=input  RightPortType=output  PseudoPeriodic=off  Frequencies=[]  NoiseDistribution=none  NoiseParameters=[]  Unit=1  AffineConversion=off  FilteringAndDerivatives=provide  SimscapeFilterOrder=1  InputFilterTimeConstant=0.001  UdotUserProvided=0
  CB : PMIOPort  Side=Right
  wires:
  [loadShutDown] -> OR/1
  Data Type Conversion1/1 -> Simulink-PS Converter2/1
  [ShutDown] -> OR/2  "System Status"
  OR/1 -> NOT/1
  NOT/1 -> Data Type Conversion1/1
  connections:
  Simulink-PS Converter2/RConn1 -- CB/RConn1

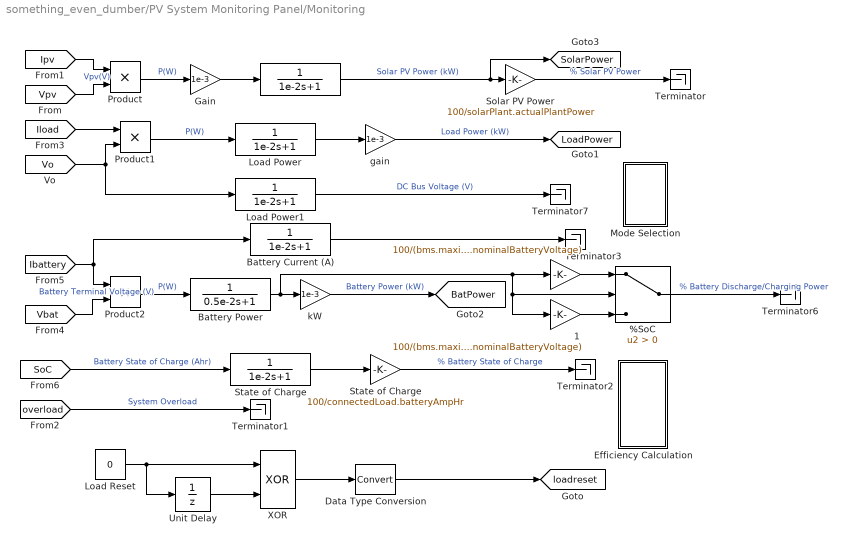
== system something_even_dumber/PV System Monitoring Panel/Monitoring ==
  " " : Gain  Gain=100/(bms.maximumChargingCurrentLimit*battery.nominalBatteryVoltage)
  "  " : TransferFcn  Denominator=[1e-2 1]
  " 1" : Gain  Gain=100/(bms.maximumDisChargingCurrent*battery.nominalBatteryVoltage)
  " State of Charge" : Gain  Gain=100/connectedLoad.batteryAmpHr
  %SoC : Switch  Criteria=u2 > Threshold  SaturateOnIntegerOverflow=off  InputSameDT=off
  Battery Current (A) : TransferFcn  Denominator=[1e-2 1]
  Battery Power : TransferFcn  Denominator=[0.5e-2 1]
  Data Type Conversion : DataTypeConversion  SaturateOnIntegerOverflow=off  RndMeth=Floor
  Efficiency Calculation : Subsystem
  Gain : Gain  Gain=1e-3
  Load Power : TransferFcn  Denominator=[1e-2 1]
  Load Power1 : TransferFcn  Denominator=[1e-2 1]
  Load Reset : Constant  Value=0
  Mode Selection : Subsystem
  Product : Product
  Product1 : Product
  Product2 : Product
  Solar PV Power : Gain  Gain=100/solarPlant.actualPlantPower
  State of Charge : TransferFcn  Denominator=[1e-2 1]
  Terminator{,1..3,6..7} (6 alike) : Terminator
  Unit Delay : UnitDelay  SampleTime=1e-3
  XOR : Logic  Operator=XOR  IconShape=distinctive  AllPortsSameDT=off  OutDataTypeStr=boolean
  gain : Gain  Gain=1e-3
  kW : Gain  Gain=1e-3
  tag scope: BatPower=global, LoadPower=global, SolarPower=global, loadreset=global
  wires:
  [Vpv] -> Product/2  "Vpv(V)"
  Load Power/1 -> gain/1
  Product1/1 -> Load Power/1  "P(W)"
  [Vbat] -> Product2/2  "Battery Terminal Voltage (V)"
  [Iload] -> Product1/1
  Battery Power/1 -> kW/1, " 1"/1, %SoC/2, " "/1
  "  "/1 -> [SolarPower], Solar PV Power/1  "Solar PV Power (kW)"
  [Ibattery] -> Product2/1, Battery Current (A)/1
  Product2/1 -> Battery Power/1  "P(W)"
  [Ipv] -> Product/1
  [Vo] -> Product1/2, Load Power1/1
  Product/1 -> Gain/1  "P(W)"
  [SoC] -> State of Charge/1  "Battery State of Charge (Ahr)"
  Solar PV Power/1 -> Terminator/1  "% Solar PV Power"
  gain/1 -> [LoadPower]  "Load Power (kW)"
  kW/1 -> [BatPower]  "Battery Power (kW)"
  State of Charge/1 -> " State of Charge"/1
  " State of Charge"/1 -> Terminator2/1  "% Battery State of Charge"
  " "/1 -> %SoC/1
  " 1"/1 -> %SoC/3
  %SoC/1 -> Terminator6/1  "% Battery Discharge/Charging Power"
  Battery Current (A)/1 -> Terminator3/1
  Gain/1 -> "  "/1
  Load Power1/1 -> Terminator7/1  "DC Bus Voltage (V)"
  [overload] -> Terminator1/1  "System Overload"
  XOR/1 -> Data Type Conversion/1
  Load Reset/1 -> XOR/1, Unit Delay/1
  Unit Delay/1 -> XOR/2
  Data Type Conversion/1 -> [loadreset]

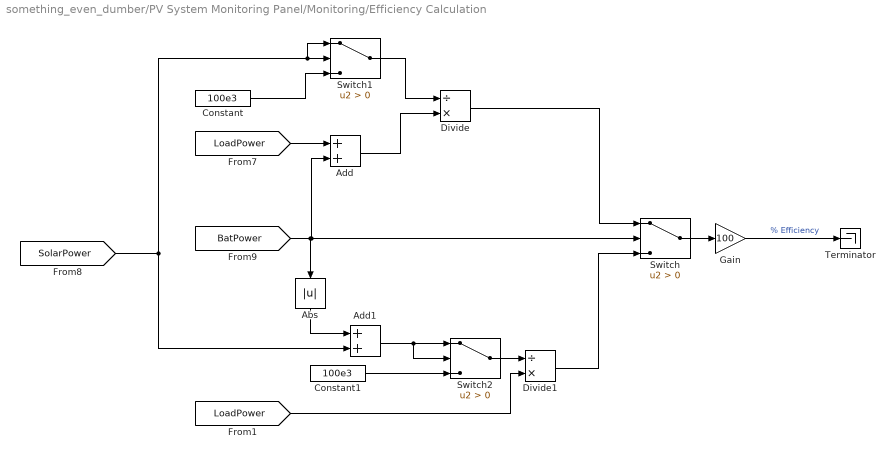
== system something_even_dumber/PV System Monitoring Panel/Monitoring/Efficiency Calculation ==
  Abs : Abs  SaturateOnIntegerOverflow=off
  Add : Sum
  Add1 : Sum
  Constant : Constant  Value=100e3
  Constant1 : Constant  Value=100e3
  Divide : Product  Inputs=/*
  Divide1 : Product  Inputs=/*
  Gain : Gain  Gain=100
  Switch : Switch  Criteria=u2 > Threshold  SaturateOnIntegerOverflow=off  InputSameDT=off
  Switch1 : Switch  Criteria=u2 > Threshold  SaturateOnIntegerOverflow=off  InputSameDT=off
  Switch2 : Switch  Criteria=u2 > Threshold  SaturateOnIntegerOverflow=off  InputSameDT=off
  Terminator : Terminator
  wires:
  [BatPower] -> Abs/1, Add/2, Switch/2
  [LoadPower] -> Add/1
  [SolarPower] -> Switch1/1, Switch1/2, Add1/2
  Constant/1 -> Switch1/3
  Switch1/1 -> Divide/1
  Add/1 -> Divide/2
  Abs/1 -> Add1/1
  [LoadPower] -> Divide1/2
  Add1/1 -> Switch2/2, Switch2/1
  Constant1/1 -> Switch2/3
  Switch2/1 -> Divide1/1
  Divide/1 -> Switch/1
  Divide1/1 -> Switch/3
  Switch/1 -> Gain/1
  Gain/1 -> Terminator/1  "% Efficiency"

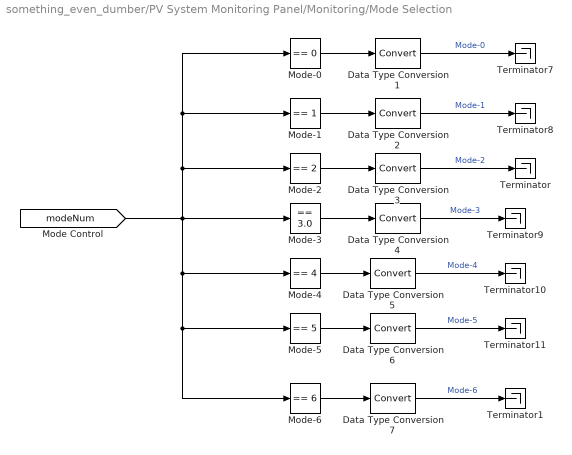
== system something_even_dumber/PV System Monitoring Panel/Monitoring/Mode Selection ==
  Data Type Conversion{1..7} (7 alike) : DataTypeConversion  SaturateOnIntegerOverflow=off  RndMeth=Floor
  Mode-0 : simulink/Logic and Bit Operations/Compare To Constant  relop===  const=0  OutDataTypeStr=boolean
  Mode-1 : simulink/Logic and Bit Operations/Compare To Constant  relop===  const=1  OutDataTypeStr=boolean
  Mode-2 : simulink/Logic and Bit Operations/Compare To Constant  relop===  const=2  OutDataTypeStr=boolean
  Mode-3 : simulink/Logic and Bit Operations/Compare To Constant  relop===  const=3.0  OutDataTypeStr=boolean
  Mode-4 : simulink/Logic and Bit Operations/Compare To Constant  relop===  const=4  OutDataTypeStr=boolean
  Mode-5 : simulink/Logic and Bit Operations/Compare To Constant  relop===  const=5  OutDataTypeStr=boolean
  Mode-6 : simulink/Logic and Bit Operations/Compare To Constant  relop===  const=6  OutDataTypeStr=boolean
  Terminator{,1,7..11} (7 alike) : Terminator
  wires:
  Mode-0/1 -> Data Type Conversion1/1
  Mode-3/1 -> Data Type Conversion4/1
  [modeNum] -> Mode-3/1, Mode-4/1, Mode-5/1, Mode-6/1, Mode-2/1, Mode-1/1, Mode-0/1
  Mode-4/1 -> Data Type Conversion5/1
  Mode-1/1 -> Data Type Conversion2/1
  Mode-2/1 -> Data Type Conversion3/1
  Mode-5/1 -> Data Type Conversion6/1
  Mode-6/1 -> Data Type Conversion7/1
  Data Type Conversion1/1 -> Terminator7/1  "Mode-0"
  Data Type Conversion2/1 -> Terminator8/1  "Mode-1"
  Data Type Conversion3/1 -> Terminator/1  "Mode-2"
  Data Type Conversion4/1 -> Terminator9/1  "Mode-3"
  Data Type Conversion5/1 -> Terminator10/1  "Mode-4"
  Data Type Conversion6/1 -> Terminator11/1  "Mode-5"
  Data Type Conversion7/1 -> Terminator1/1  "Mode-6"

== matlab function something_even_dumber/PV_MPPT_6module ==
  settings: updateMethod=DISCRETE
  data: G input; Ibus output; T input; Vbus input; en input; VmpT input; ImpT input; Pbus output; Pavail output; Vpv output; Ipv output; Imod output; duty output
function [Ibus, Pbus, Pavail, Vpv, Ipv, Imod, duty] = fcn(G,T,Vbus,en,VmpT,ImpT)
%#codegen
% EOL teammate MPP data; illustrative piecewise I-V fit.
% Shared PV bus, single coordinated P&O, six averaged PI branches.
persistent Vcmd dir Pprev count il integ
if isempty(Vcmd)
 Vcmd=217; dir=1; Pprev=0; count=0; il=zeros(6,1); integ=zeros(6,1);
end
dt=1e-4; eta=0.96; Gref=1367;
gs=max(0,min(1.5,G/Gref));
vmp=max(10,VmpT); imp=max(0,ImpT)*gs;
% Curve passes through Isc, Imp at Vmp, and zero at Voc.
% Isc=1.04 Imp, Voc=1.13 Vmp are MODEL ASSUMPTIONS.
isc=1.04*imp; voc=1.13*vmp;
Vcmd=max(0.5*vmp,min(0.99*voc,Vcmd));
if Vcmd<=vmp
 ipv=max(0,isc-(isc-imp)*(Vcmd/vmp)^2);
else
 ipv=max(0,imp*(voc-Vcmd)/(voc-vmp));
end
Ppv=Vcmd*ipv; Pavail=max(0,vmp*imp*eta);
count=count+1;
if count>=100
 if Ppv<Pprev, dir=-dir; end
 Vcmd=Vcmd+dir*0.5; Pprev=Ppv; count=0;
end
% Power-to-current reference; current limited by PV production.
v=max(30,Vbus);
Ptarget=max(0,min(Ppv*eta,Pavail))*max(0,min(1,en));
Iref=Ptarget/v/6;
Imod=zeros(6,1); duty=zeros(6,1);
for k=1:6
 % Averaged current PI with feedforward; shared-array duty proxy.
 err=Iref-il(k);
 dff=Vbus/max(1,1.15*Vcmd);
 d=max(0,min(0.85,dff+0.0015*err+integ(k)));
 % Average inductor dynamics; 33 uH each.
 next=il(k)+dt*(1.15*Vcmd*d-Vbus)/33e-6;
 % Avoid nonphysical reverse PV current.
 next=max(0,next);
 % Anti-windup: integrate only when unsaturated or correcting.
 if (d>0 && d<0.85) || (d<=0 && err>0) || (d>=0.85 && err<0)
  integ(k)=integ(k)+3*dt*err;
 end
 il(k)=next; Imod(k)=next; duty(k)=d;
end
% Conservation clamp: do not inject more power than PV can supply.
Iraw=sum(Imod); Ibus=min(Iraw,Ptarget/v);
Pbus=Ibus*max(0,Vbus); Vpv=Vcmd; Ipv=ipv;
end

== stateflow chart something_even_dumber/Mode Control ==
  state Mode2_BatCharge_pvMPPT
    entry:
    pvMPPT=1;
    BatCharge=1;
    modeNum=2;
    overload=0;
    exit:
    pvMPPT=0; BatCharge=0;
  state Start_Mode
    entry:
    ShutDown = 0;
    loadShutDown = 1;
    pvMPPT=0;
    VoltageControl=1;
    BatIsolate=1;
    modeNum=0;
    overload=0;
    exit:
    pvMPPT=0;
    BatIsolate=0;
    VoltageControl=0;
    loadShutDown = 0;
  state Mode5_System_ShutDown
    entry:
    PVoff=1; BatIsolate=1;
    ShutDown =1; modeNum=5;
    exit:
    ShutDown =0; PVoff=0;
    BatIsolate=0;
  state Mode1_batIsolated_pvVoltControl
    entry:
    VoltageControl=1; BatIsolate=1;
    modeNum=1;
    exit:
    VoltageControl=0; BatIsolate=0;
  state Mode6_pvMPPT_BatCharge_noload
    entry:
    pvMPPT=1; BatCharge=1;
    loadShutDown=1; modeNum=6;
    overload=1;
    exit:
    loadShutDown=0; pvMPPT=0;
    BatCharge=0;
  state Mode3_BatDischarge_pvMPPT
    entry:
    pvMPPT=1; BatDischarge=1;
    modeNum=3; overload=0;
    exit:
    pvMPPT=0;  BatDischarge=0;
  state Mode4_night_mode
    entry:
    PVoff=1; BatDischarge=1;
    modeNum=4;
    exit:
    PVoff=0; BatDischarge=0;
  Mode2_BatCharge_pvMPPT -> (junction 121) [order 3] : [Irrad<minIrrad && SoC>minSoC]
  Mode2_BatCharge_pvMPPT -> (junction 131) [order 2] : [Vdc < minVdc && SoC>minSoC]
  (junction 121) -> Mode4_night_mode
  (junction 131) -> (junction 154)
  Mode2_BatCharge_pvMPPT -> (junction 117) [order 5] : [Irrad<minIrrad && SoC<minSoC]
  (junction 132) -> Mode2_BatCharge_pvMPPT : [Vdc > maxVdc && Irrad>minIrrad]
  (junction 117) -> Mode5_System_ShutDown
  (junction 155) -> (junction 132)
  (junction 130) -> Mode2_BatCharge_pvMPPT : [(Irrad >minIrrad && overload==0) || ...
      | (overload==1 && rsflag==1)]
  Mode5_System_ShutDown -> (junction 130)
  Start_Mode -> Mode2_BatCharge_pvMPPT [order 1] : [SoC<minSoC]
  (junction 123) -> Mode2_BatCharge_pvMPPT
  Mode6_pvMPPT_BatCharge_noload -> (junction 123) [order 3] : [rsflag ==1 && Irrad > minIrrad  ...
      | && SoC <= minSoC]
  Mode2_BatCharge_pvMPPT -> (junction 125) [order 4]
  (default) -> Start_Mode
  (junction 125) -> Mode6_pvMPPT_BatCharge_noload : [duration(Vdc<minVdc)>olTime ...
      |  && SoC<minSoC]
  Mode2_BatCharge_pvMPPT -> Mode1_batIsolated_pvVoltControl [order 1] : [(SoC>maxSoC) || ...
      | (duration(Vdc>maxVdc)>olTime)]
  Start_Mode -> Mode3_BatDischarge_pvMPPT [order 2] : [SoC>minSoC]
  Mode1_batIsolated_pvVoltControl -> (junction 126)
  Mode6_pvMPPT_BatCharge_noload -> Mode5_System_ShutDown [order 2] : [(SoC<minSoC && ...
      | Irrad<minIrrad)|| ...
      | SoC>maxSoC]
  (junction 126) -> Mode3_BatDischarge_pvMPPT : [Vdc<minVdc]
  (junction 161) -> Mode5_System_ShutDown
  Mode4_night_mode -> Mode5_System_ShutDown [order 2] : [SoC<minSoC]
  Mode6_pvMPPT_BatCharge_noload -> (junction 127) [order 1] : [SoC>minSoC && rsflag==1]
  (junction 127) -> Mode3_BatDischarge_pvMPPT
  (junction 133) -> Mode6_pvMPPT_BatCharge_noload
  Mode3_BatDischarge_pvMPPT -> (junction 133) [order 2] : [(duration(Vdc<minVdc)>olTime || ...
      |  (SoC<minSoC && Vdc<minVdc)) && Irrad>minIrrad]
  Mode3_BatDischarge_pvMPPT -> (junction 161) [order 3] : [(SoC<minSoC && Irrad<minIrrad) || ( Irrad<minIrrad && duration(Vdc<minVdc)>olTime) ]
  Mode3_BatDischarge_pvMPPT -> (junction 155) [order 1]
  Mode4_night_mode -> Mode3_BatDischarge_pvMPPT [order 1] : [Irrad>minIrrad]
  Mode3_BatDischarge_pvMPPT -> Mode4_night_mode [order 4] : [Irrad<minIrrad && SoC>minSoC]
  (junction 154) -> Mode3_BatDischarge_pvMPPT
  data: Irrad input; Vdc input; SoC input; ShutDown output; maxSoC parameter; maxVdc parameter; minIrrad parameter; minSoC parameter; minVdc parameter; loadShutDown output; VoltageControl output; BatCharge output; BatDischarge output; BatIsolate output; PVoff output; pvMPPT output; modeNum output; rsflag input; overload output; olTime parameter
